simulink model "Slope_Road_SideSlipAngle_Vx_Estimation"  (R2024b)
settings: Solver=FixedStepAuto  StartTime=0.0  StopTime=7.5  FixedStep=0.001  RelTol=1e-4
values from neighbouring files (symbols this model uses):
  ax_long_1 = 1    [Init.m]
  ax_long_2 = 3    [Init.m]
  ax_long_3 = 6    [Init.m]
  ax_steer_1 = 0.5    [Init.m]
  ax_steer_2 = 1.5    [Init.m]
  ax_steer_3 = 3    [Init.m]
  ax_vx_thres1 = 0.5    [Init.m]
  ax_vx_thres2 = 3    [Init.m]
  Brush = [28.93,1.496,0.9486,0.06054]    [Init.m]
  delay_constant = 1/delay_length*ones(1,round(delay_length))    [Init.m]
  delta_thres = 3*3.14/180    (= 0.0523333333333)    [Init.m]
  deltarate_thres = 0.1    [Init.m]
  dg2rd = pi/180    (= 0.0174532925199)    [Init.m]
  excessive_wheel_intgr = 1000    [Init.m]
  filter_ratio_ax_ay = 0.2    [Init.m]
  g = 9.8    [Init.m]
  gao_ay = 1.5    [Init.m]
  gao_D_v = 0.2    [Init.m]
  gao_D_w = 0.03    [Init.m]
  gao_D_w1 = 0.25    [Init.m]
  gao_gz = 0.1    [Init.m]
  gao_Q = 1e-02    (= 0.01)    [Init.m]
  gao_R = 0.00077574*0.1    (= 7.7574e-05)    [Init.m]
  K_theta = 1    [Init.m]
  k_vx_vari_thres1 = 20    [Init.m]
  k_vx_vari_thres2 = 20    [Init.m]
  k_vx_vari_thres3 = 20    [Init.m]
  k_vy = 1/veh_m0    (= 0.000327653997379)    [Init.m]
  N_num = 6    [Init.m]
  para_long_1 = 1    [Init.m]
  para_long_2 = 100    [Init.m]
  para_long_3 = 100000000    [Init.m]
  para_long_4 = 100    [Init.m]
  para_steer_1 = 0.1    [Init.m]
  para_steer_2 = 10    [Init.m]
  para_steer_3 = 1000    [Init.m]
  para_steer_4 = 1000    [Init.m]
  rd2dg = 180/pi    (= 57.2957795131)    [Init.m]
  Steer_angle = 0    [Init.m]
  tao_1 = 6    [Init.m]
  time_interval = 1/Ts    (= 1000)    [Init.m]
  Ts = 0.001    [Init.m]
  u_init = 0.9    [Init.m]
  veh_bf = 1.600    (= 1.6)    [Init.m]
  veh_br = 1.740    (= 1.74)    [Init.m]
  veh_lf = 1.293    [Init.m]
  veh_lr = veh_l-veh_lf    (= 1.835)    [Init.m]
  veh_m0 = 3052    [Init.m]
  vx_cri = 1    [Init.m]
  vx_lowest = 0.01    [Init.m]
  vx_max_diff = 1    [Init.m]
  vy_new_ini = 0    [Init.m]
  wh_r = 0.346    [Init.m]
undefined symbols (not defined in the file or in its folder): DiscIntNeverNeededParam, front_gear_ratio, rear_gear_ratio, steer_ratio
libraries: simulink x7, Solver_SF x1
(part 1 of 2)
settings Model: Creator=Lenovo  LastModifiedBy=13785
settings SolverCC: AlgebraicLoopSolver=TrustRegion
settings OptimizationCC: LifeSpan=inf
settings DebuggingCC: UnconnectedInputMsg=warning  UnconnectedOutputMsg=warning  UnconnectedLineMsg=warning  SFExecutionAtInitializationDiag=none  ArithmeticOperatorsInVariantConditions=warning
settings ModelReferenceCC: EnableRefExpFcnMdlSchedulingChecks=on
settings SFSimCC: CustomCodeUndefinedFunction=UseInterfaceOnly
settings RTWCC: GPUComputeCapability=3.5
settings CodeAppCC: StateflowObjectComments=on

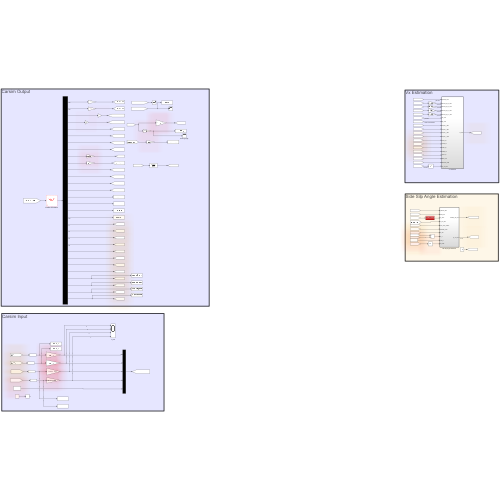
[thumbnail: Simulink's stored preview of the top-level diagram]
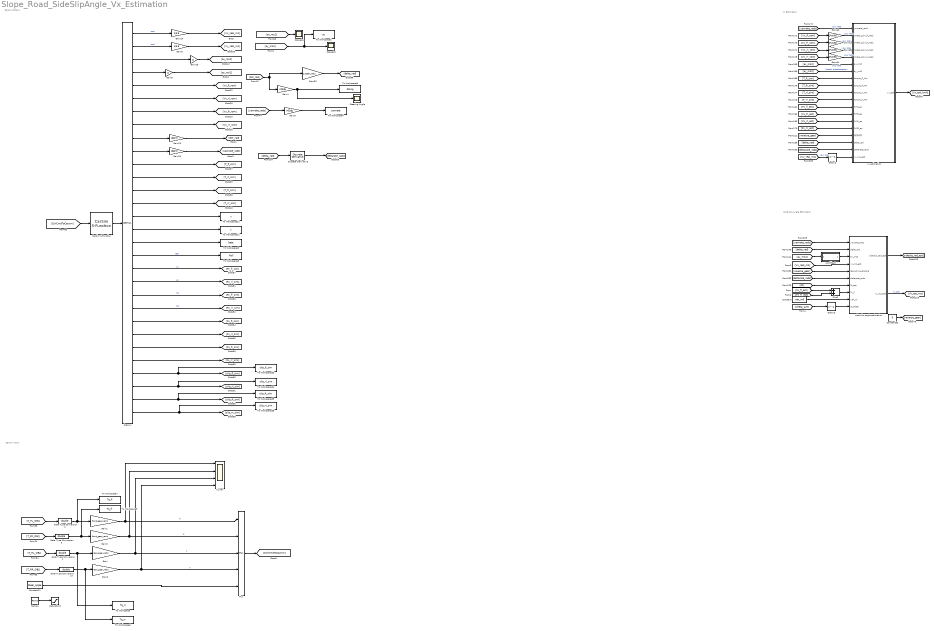
== system Slope_Road_SideSlipAngle_Vx_Estimation ==
  note: Vx Estimation
  note: Side Silp Angle Estimation
  note: Carsim Input
  note: Carsim Output
  CarSim S-Function : Solver_SF/CarSim S-Function  Priority=1  SIMFILE=simfile.sim  Run_RTs=off  vs_state_ind=Run  StopMode_ind=Vehicle Model
  Constant : Constant  Value=veh_m0
  Constant11 : Constant  Value=Steer_angle
  Constant32 : Constant  Value=0
  Data Type Conversion{1..3,27} (4 alike) : DataTypeConversion  OutDataTypeStr=double  SaturateOnIntegerOverflow=off  RndMeth=Floor
  Delay2 : Delay  DelayLength=1
  Delay3 : Delay  DelayLength=1  InitialCondition=u_init
  Demux : Demux  Outputs=30
  Discrete Derivative : simulink/Discrete/Discrete Derivative  gainval=1.0  ICPrevScaledInput=0.0  OutMin=[]  OutMax=[]  OutDataType=fixdt(1, 16)  OutScaling=2^-10  DoSatur=off
  Gain : Gain  Gain=rear_gear_ratio
  Gain1 : Gain  Gain=front_gear_ratio
  Gain2 : Gain  Gain=rear_gear_ratio
  Gain24 : Gain  Gain=1/3.6
  Gain25 : Gain  Gain=dg2rd
  Gain26 : Gain  Gain=dg2rd
  Gain29 : Gain  Gain=g
  Gain3 : Gain  Gain=front_gear_ratio
  Gain4 : Gain  Gain=rd2dg
  Gain5 : Gain  Gain=rd2dg
  Gain53 : Gain  Gain=1/steer_ratio
  Gain6 : Gain  Gain=1/3.6
  Gain{60..61,63..64} (4 alike) : Gain  Gain=2*pi/60
  Gain8 : Gain  Gain=g
  Mux : Mux  Inputs=5
  Plus2 : Sum
  Ramp1 : simulink/Sources/Ramp  slope=500  start=1  InitialOutput=0
  Saturation1 : Saturate  UpperLimit=300
  Scope10 : Scope
  Scope16 : Scope
  Steering Angle : Scope
  T_final : Scope  NumInputPorts=4
  To Workspace : ToWorkspace  VariableName=Tq_rl  SaveFormat=Timeseries  SampleTime=-1
  To Workspace11 : ToWorkspace  VariableName=x  SaveFormat=Timeseries  SampleTime=-1
  To Workspace12 : ToWorkspace  VariableName=y  SaveFormat=Timeseries  SampleTime=-1
  To Workspace2 : ToWorkspace  VariableName=ay  SaveFormat=Timeseries  SampleTime=-1
  To Workspace3 : ToWorkspace  VariableName=StAng  SaveFormat=Timeseries  SampleTime=-1
  To Workspace33 : ToWorkspace  VariableName=slip_fl_sim  SaveFormat=Timeseries  SampleTime=-1
  To Workspace34 : ToWorkspace  VariableName=slip_rl_sim  SaveFormat=Timeseries  SampleTime=-1
  To Workspace35 : ToWorkspace  VariableName=slip_fr_sim  SaveFormat=Timeseries  SampleTime=-1
  To Workspace36 : ToWorkspace  VariableName=slip_rr_sim  SaveFormat=Timeseries  SampleTime=-1
  To Workspace4 : ToWorkspace  VariableName=yawrate  SaveFormat=Timeseries  SampleTime=-1
  To Workspace5 : ToWorkspace  VariableName=beta  SaveFormat=Timeseries  SampleTime=-1
  To Workspace6 : ToWorkspace  VariableName=Tq_rr  SaveFormat=Timeseries  SampleTime=-1
  To Workspace7 : ToWorkspace  VariableName=Tq_fl  SaveFormat=Timeseries  SampleTime=-1
  To Workspace8 : ToWorkspace  VariableName=Roll  SaveFormat=Timeseries  SampleTime=-1
  To Workspace9 : ToWorkspace  VariableName=Tq_fr  SaveFormat=Timeseries  SampleTime=-1
  rpmfilter3 : Subsystem
  "side slip angle estimation " : Subsystem  TreatAsAtomicUnit=on
  vx estimation : Subsystem  TreatAsAtomicUnit=on
  wires:
  "side slip angle estimation "/2(vy_ms_esti) -> [Vy_est_ms]  "vy_est"
  [Fx_fl_est] -> Plus2/1
  [yawrate_rads] -> "side slip angle estimation "/1(yawrate_rads)
  Plus2/1 -> "side slip angle estimation "/8(Fx_f)
  [reverse_gear] -> "side slip angle estimation "/5(rear_drive_enable)
  [Fx_fr_est] -> Plus2/2
  "side slip angle estimation "/1(sideslip_rad_esti) -> [sideslip_rad_esti]
  [Fz] -> "side slip angle estimation "/7(Fz_est)
  [delta_rad] -> "side slip angle estimation "/2(delta_rad)
  rpmfilter3/1(fliter_out) -> "side slip angle estimation "/3(ay_ms2)
  [deltarate_rads] -> "side slip angle estimation "/6(deltarate_rads)
  [ay_ms2] -> rpmfilter3/1(fliter_in)
  Constant/1 -> "side slip angle estimation "/9(veh_m)
  Delay3/1 -> "side slip angle estimation "/10(rd_theta)
  Constant32/1 -> [reverse_gear]
  [deltarate_rads] -> vx estimation/18(deltarate_rads)
  [Vx_rl_rpm] -> Gain63/1
  Gain61/1 -> vx estimation/3(wheel_spin_fr_rads)  "yaw rate"
  Delay2/1 -> vx estimation/19(vy_ms_esti)
  [T_rl_sim] -> vx estimation/10(torque_rl_Nm)
  [Fx_fr_est] -> vx estimation/13(FxFR_es)
  [Vy_real_ms] -> Delay2/1  "yaw rate"
  [Vx_fr_rpm] -> Gain61/1
  [T_fl_sim] -> vx estimation/8(torque_fl_Nm)
  [Vx_fl_rpm] -> Gain60/1
  Gain63/1 -> vx estimation/4(wheel_spin_rl_rads)  "yaw rate"
  [reverse_gear] -> vx estimation/16(倒挡信息)
  [yawrate_rads] -> vx estimation/1(yawrate_rads)  "yaw rate"
  Gain64/1 -> vx estimation/5(wheel_spin_rr_rads)  "yaw rate"
  Gain60/1 -> vx estimation/2(wheel_spin_fl_rads)  "yaw rate"
  [ax_ms2] -> vx estimation/6(ax_ms2)  "yaw rate"
  [delta_rad] -> vx estimation/17(delta_rad)
  vx estimation/1(vx_esti) -> [Vx_est_kmh]
  [Fx_fl_est] -> vx estimation/12(FxFL_es)
  [ay_ms2] -> vx estimation/7(ay_ms2)  "lateral acceleratation"
  [Fx_rr_est] -> vx estimation/15(FxRR_es)
  [T_rr_sim] -> vx estimation/11(torque_rr_Nm)
  [Fx_rl_est] -> vx estimation/14(FxRL_es)
  [Vx_rr_rpm] -> Gain64/1
  [T_fr_sim] -> vx estimation/9(torque_fr_Nm)
  [Vx_real_ms] -> "side slip angle estimation "/4(vx_ms_esti)
  [theta_ave] -> Delay3/1
  Gain29/1 -> [ax_ms2]
  Gain1/1 -> T_final/1, Mux/1  "fl"
  Demux/2 -> Gain6/1  "real"
  Demux/26 -> [Fx_rr_sim]
  [CtrlCmdToCarsim] -> CarSim S-Function/1
  Demux/12 -> [T_rl_sim]
  Demux/5 -> [Vx_fl_rpm]
  [ax_ms2] -> Scope16/1
  [delta_rad] -> Discrete Derivative/1
  Gain5/1 -> To Workspace4/1
  CarSim S-Function/1 -> Demux/1
  Demux/7 -> [Vx_fr_rpm]
  [T_FR_OBJ] -> Data Type Conversion3/1
  Demux/30 -> [slip_rr_sim], To Workspace36/1
  Demux/11 -> [T_fl_sim]
  Mux/1 -> [CtrlCmdToCarsim]
  Demux/10 -> Gain26/1
  Gain26/1 -> [yawrate_rads]
  Data Type Conversion27/1 -> To Workspace6/1, Gain2/1
  Demux/29 -> [slip_fr_sim], To Workspace35/1
  Demux/4 -> Gain8/1
  [ay_ms2] -> Scope10/1, To Workspace2/1
  Gain8/1 -> [ay_ms2]
  Gain3/1 -> Mux/2, T_final/2  "fr"
  Demux/27 -> To Workspace33/1, [slip_fl_sim]
  Demux/1 -> Gain24/1  "real"
  Gain4/1 -> Steering Angle/1, To Workspace3/1
  Gain6/1 -> [Vy_real_ms]
  Data Type Conversion1/1 -> To Workspace/1, Gain/1
  Demux/28 -> [slip_rl_sim], To Workspace34/1
  Demux/9 -> Gain25/1
  Demux/8 -> [Vx_rr_rpm]
  Gain/1 -> Mux/3, T_final/3  "rl"
  Constant11/1 -> Mux/5
  Data Type Conversion2/1 -> To Workspace7/1, Gain1/1
  Demux/13 -> [T_fr_sim]
  [T_RL_OBJ] -> Data Type Conversion1/1
  [T_RR_OBJ] -> Data Type Conversion27/1
  Demux/3 -> Gain29/1
  Gain24/1 -> [Vx_real_ms]
  Demux/6 -> [Vx_rl_rpm]
  Gain2/1 -> Mux/4, T_final/4  "rr"
  Gain25/1 -> [SW_rad]
  Demux/14 -> [T_rr_sim]
  Gain53/1 -> [delta_rad]
  Discrete Derivative/1 -> [deltarate_rads]
  [SW_rad] -> Gain4/1, Gain53/1
  Data Type Conversion3/1 -> To Workspace9/1, Gain3/1
  Ramp1/1 -> Saturation1/1
  [yawrate_rads] -> Gain5/1
  [T_FL_OBJ] -> Data Type Conversion2/1
  Demux/19 -> [Fz_fl_sim]  "L1"
  Demux/20 -> [Fz_rl_sim]  "L2"
  Demux/21 -> [Fz_fr_sim]  "R1"
  Demux/22 -> [Fz_rr_sim]  "R2"
  Demux/25 -> [Fx_fr_sim]
  Demux/24 -> [Fx_rl_sim]
  Demux/23 -> [Fx_fl_sim]
  Demux/15 -> To Workspace11/1
  Demux/16 -> To Workspace12/1
  Demux/17 -> To Workspace5/1
  Demux/18 -> To Workspace8/1  "real"

== system Slope_Road_SideSlipAngle_Vx_Estimation/rpmfilter3 ==
  fliter_in : Inport
  Constant1 : Constant  OutDataTypeStr=single
  Divide : Product  Inputs=**
  Divide1 : Product  Inputs=**
  Sum : Sum  Inputs=|-+
  Sum1 : Sum  Inputs=|++
  Unit Delay : UnitDelay  SampleTime=-1  HasFrameUpgradeWarning=on
  afa : Constant  Value=filter_ratio_ax_ay  OutDataTypeStr=single
  fliter_out : Outport
  wires:
  Unit Delay/1 -> Divide1/2
  fliter_in/1 -> Divide/1
  Divide1/1 -> Sum1/2
  Divide/1 -> Sum1/1
  Sum/1 -> Divide1/1
  afa/1 -> Divide/2, Sum/1
  Constant1/1 -> Sum/2
  Sum1/1 -> Unit Delay/1, fliter_out/1

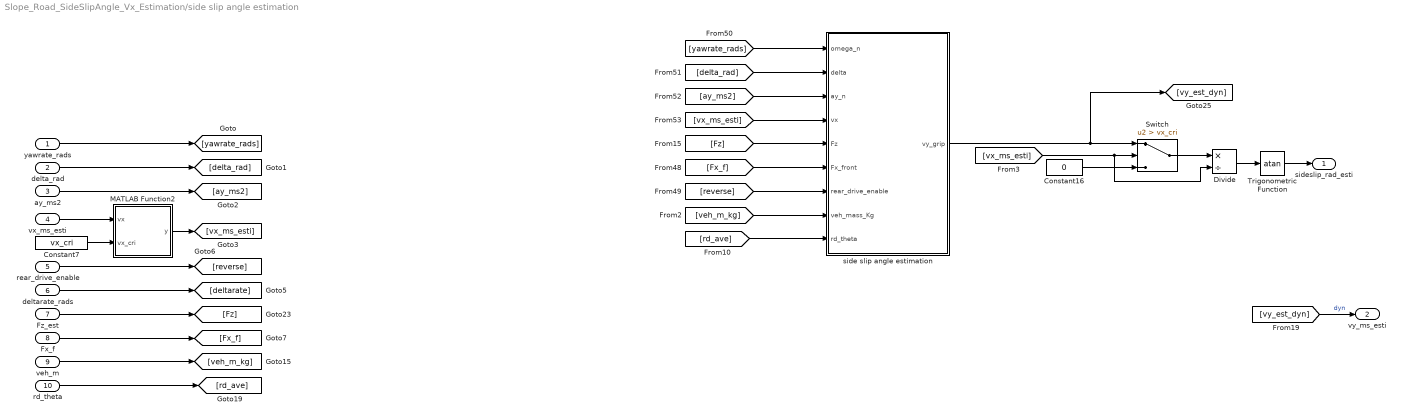
== system Slope_Road_SideSlipAngle_Vx_Estimation/side slip angle estimation  ==
  yawrate_rads : Inport
  delta_rad : Inport  Port=2
  ay_ms2 : Inport  Port=3
  vx_ms_esti : Inport  Port=4
  rear_drive_enable : Inport  Port=5
  deltarate_rads : Inport  Port=6
  Fz_est : Inport  Port=7
  Fx_f : Inport  Port=8
  veh_m : Inport  Port=9
  rd_theta : Inport  Port=10
  Constant16 : Constant  Value=0
  Constant7 : Constant  Value=vx_cri
  Divide : Product  Inputs=*/
  MATLAB Function2 : MATLAB Function  TreatAsAtomicUnit=on
  Switch : Switch  Criteria=u2 > Threshold  Threshold=vx_cri  SaturateOnIntegerOverflow=off  InputSameDT=off
  Trigonometric Function : Trigonometry  Operator=atan
  side slip angle estimation : Subsystem  TreatAsAtomicUnit=on
  sideslip_rad_esti : Outport
  vy_ms_esti : Outport  Port=2
  wires:
  vx_ms_esti/1 -> MATLAB Function2/1(vx)
  MATLAB Function2/1(y) -> [vx_ms_esti]
  Constant7/1 -> MATLAB Function2/2(vx_cri)
  ay_ms2/1 -> [ay_ms2]
  yawrate_rads/1 -> [yawrate_rads]
  delta_rad/1 -> [delta_rad]
  Fz_est/1 -> [Fz]
  deltarate_rads/1 -> [deltarate]
  Fx_f/1 -> [Fx_f]
  veh_m/1 -> [veh_m_kg]
  rear_drive_enable/1 -> [reverse]
  rd_theta/1 -> [rd_ave]
  [yawrate_rads] -> side slip angle estimation/1(omega_n)
  [Fx_f] -> side slip angle estimation/6(Fx_front)
  [delta_rad] -> side slip angle estimation/2(delta)
  [vx_ms_esti] -> side slip angle estimation/4(vx)
  [ay_ms2] -> side slip angle estimation/3(ay_n)
  [Fz] -> side slip angle estimation/5(Fz)
  Constant16/1 -> Switch/3
  side slip angle estimation/1(vy_grip) -> [vy_est_dyn], Switch/1
  [vx_ms_esti] -> Divide/2, Switch/2
  Switch/1 -> Divide/1
  [veh_m_kg] -> side slip angle estimation/8(veh_mass_Kg)
  Trigonometric Function/1 -> sideslip_rad_esti/1
  [rd_ave] -> side slip angle estimation/9(rd_theta)
  Divide/1 -> Trigonometric Function/1
  [vy_est_dyn] -> vy_ms_esti/1  "dyn"
  [reverse] -> side slip angle estimation/7(rear_drive_enable)

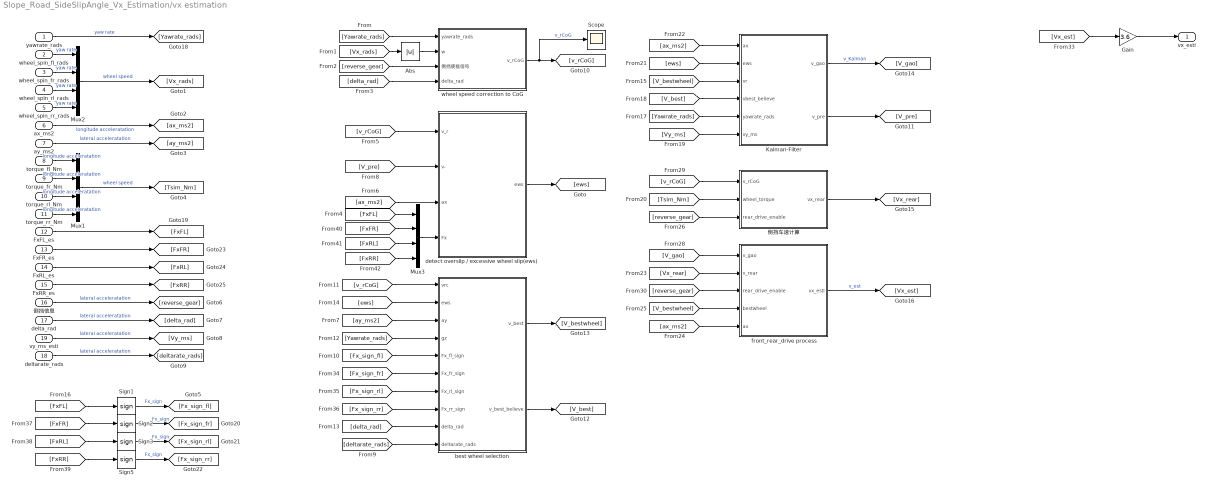
== system Slope_Road_SideSlipAngle_Vx_Estimation/vx estimation ==
  yawrate_rads : Inport
  wheel_spin_fl_rads : Inport  Port=2
  wheel_spin_fr_rads : Inport  Port=3
  wheel_spin_rl_rads : Inport  Port=4
  wheel_spin_rr_rads : Inport  Port=5
  ax_ms2 : Inport  Port=6
  ay_ms2 : Inport  Port=7
  torque_fl_Nm : Inport  Port=8
  torque_fr_Nm : Inport  Port=9
  torque_rl_Nm : Inport  Port=10
  torque_rr_Nm : Inport  Port=11
  FxFL_es : Inport  Port=12
  FxFR_es : Inport  Port=13
  FxRL_es : Inport  Port=14
  FxRR_es : Inport  Port=15
  倒挡信息 : Inport  Port=16
  delta_rad : Inport  Port=17
  deltarate_rads : Inport  Port=18
  vy_ms_esti : Inport  Port=19
  Abs : Abs  SaturateOnIntegerOverflow=off
  Gain : Gain  Gain=3.6
  Kalman-Filter : Subsystem
  Mux1 : Mux
  Mux2 : Mux
  Mux3 : Mux
  Scope : Scope
  Sign{1..3,5} (4 alike) : Signum
  "best wheel selection " : Subsystem
  detect overslip / excessive wheel slip(ews) : Subsystem
  front_rear_drive process : Subsystem  TreatAsAtomicUnit=on
  wheel speed correction to CoG : Subsystem
  倒挡车速计算 : Subsystem  TreatAsAtomicUnit=on
  vx_esti : Outport
  wires:
  vy_ms_esti/1 -> [Vy_ms]  "lateral acceleratation"
  torque_rr_Nm/1 -> Mux1/4  "longitude acceleratation"
  torque_rl_Nm/1 -> Mux1/3  "longitude acceleratation"
  torque_fr_Nm/1 -> Mux1/2  "longitude acceleratation"
  torque_fl_Nm/1 -> Mux1/1  "longitude acceleratation"
  wheel_spin_rr_rads/1 -> Mux2/4  "yaw rate"
  wheel_spin_rl_rads/1 -> Mux2/3  "yaw rate"
  wheel_spin_fr_rads/1 -> Mux2/2  "yaw rate"
  wheel_spin_fl_rads/1 -> Mux2/1  "yaw rate"
  yawrate_rads/1 -> [Yawrate_rads]  "yaw rate"
  Mux2/1 -> [Vx_rads]  "wheel speed"
  ax_ms2/1 -> [ax_ms2]  "longitude acceleratation"
  ay_ms2/1 -> [ay_ms2]  "lateral acceleratation"
  Mux1/1 -> [Tsim_Nm]  "wheel speed"
  FxFL_es/1 -> [FxFL]
  倒挡信息/1 -> [reverse_gear]  "lateral acceleratation"
  delta_rad/1 -> [delta_rad]  "lateral acceleratation"
  deltarate_rads/1 -> [deltarate_rads]  "lateral acceleratation"
  [Vx_rads] -> Abs/1
  [Yawrate_rads] -> wheel speed correction to CoG/1(yawrate_rads)
  wheel speed correction to CoG/1(v_rCoG) -> Scope/1, [v_rCoG]  "v_rCoG"
  [delta_rad] -> wheel speed correction to CoG/4(delta_rad)
  [reverse_gear] -> wheel speed correction to CoG/3(倒挡使能信号)
  Abs/1 -> wheel speed correction to CoG/2(w)
  [v_rCoG] -> detect overslip / excessive wheel slip(ews)/1(v_r)
  [ax_ms2] -> detect overslip / excessive wheel slip(ews)/3(ax)
  [V_pre] -> detect overslip / excessive wheel slip(ews)/2(v-)
  detect overslip / excessive wheel slip(ews)/1(ews) -> [ews]
  "best wheel selection "/2(v_best_believe) -> [V_best]
  [v_rCoG] -> "best wheel selection "/1(vrc)
  "best wheel selection "/1(v_best) -> [V_bestwheel]
  [Yawrate_rads] -> "best wheel selection "/4(gz)
  [delta_rad] -> "best wheel selection "/9(delta_rad)
  [deltarate_rads] -> "best wheel selection "/10(deltarate_rads)
  [ay_ms2] -> "best wheel selection "/3(ay)
  [ews] -> "best wheel selection "/2(ews)
  [Yawrate_rads] -> Kalman-Filter/5(yawrate_rads)
  [Vy_ms] -> Kalman-Filter/6(vy_ms)
  [V_bestwheel] -> Kalman-Filter/3(vr)
  [ax_ms2] -> Kalman-Filter/1(ax)
  [V_best] -> Kalman-Filter/4(vbest_believe)
  [ews] -> Kalman-Filter/2(ews)
  Kalman-Filter/2(v_pre) -> [V_pre]
  Kalman-Filter/1(v_gao) -> [V_gao]  "v_Kalman"
  [reverse_gear] -> 倒挡车速计算/3(rear_drive_enable)
  [v_rCoG] -> 倒挡车速计算/1(v_rCoG)
  [ax_ms2] -> front_rear_drive process/5(ax)
  [reverse_gear] -> front_rear_drive process/3(rear_drive_enable)
  [Tsim_Nm] -> 倒挡车速计算/2(wheel_torque)
  [V_bestwheel] -> front_rear_drive process/4(bestwheel)
  [V_gao] -> front_rear_drive process/1(v_gao)
  倒挡车速计算/1(vx_rear) -> [Vx_rear]
  [Vx_rear] -> front_rear_drive process/2(v_rear)
  front_rear_drive process/1(vx_esti) -> [Vx_est]  "v_est"
  [Vx_est] -> Gain/1
  Gain/1 -> vx_esti/1
  Mux3/1 -> detect overslip / excessive wheel slip(ews)/4(Fx)
  Sign1/1 -> [Fx_sign_fl]  "Fx_sign"
  Sign2/1 -> [Fx_sign_fr]  "Fx_sign"
  Sign3/1 -> [Fx_sign_rl]  "Fx_sign"
  Sign5/1 -> [Fx_sign_rr]  "Fx_sign"
  [Fx_sign_fl] -> "best wheel selection "/5(Fx_fl_sign)
  [Fx_sign_fr] -> "best wheel selection "/6(Fx_fr_sign)
  [Fx_sign_rl] -> "best wheel selection "/7(Fx_rl_sign)
  [Fx_sign_rr] -> "best wheel selection "/8(Fx_rr_sign)
  FxFR_es/1 -> [FxFR]
  FxRL_es/1 -> [FxRL]
  FxRR_es/1 -> [FxRR]
  [FxFL] -> Sign1/1
  [FxFR] -> Sign2/1
  [FxRL] -> Sign3/1
  [FxRR] -> Sign5/1
  [FxFR] -> Mux3/2
  [FxFL] -> Mux3/1
  [FxRL] -> Mux3/3
  [FxRR] -> Mux3/4

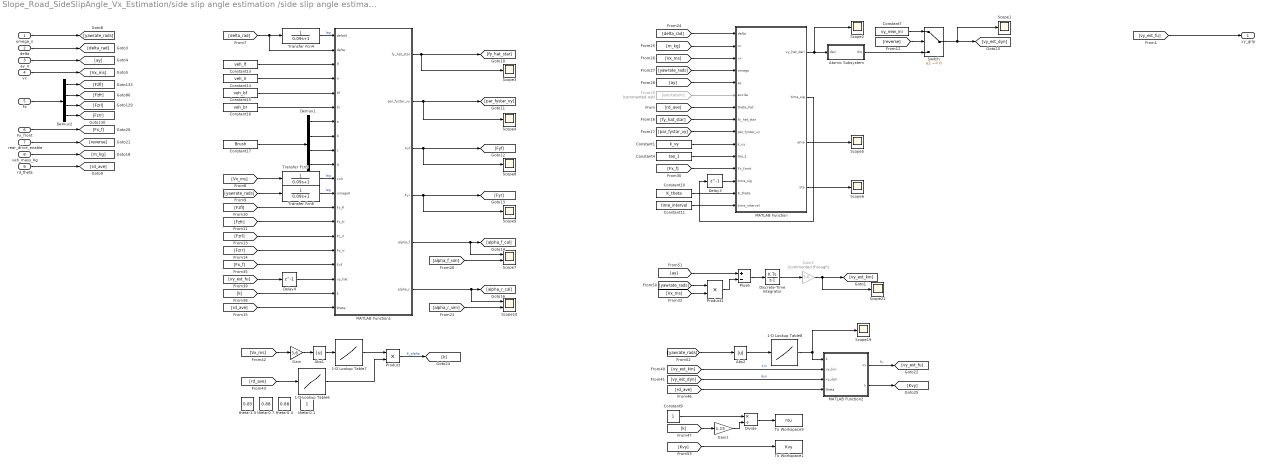
== system Slope_Road_SideSlipAngle_Vx_Estimation/side slip angle estimation /side slip angle estimation ==
  omega_n : Inport
  delta : Inport  Port=2
  ay_n : Inport  Port=3
  vx : Inport  Port=4
  Fz : Inport  Port=5
  Fx_front : Inport  Port=6
  rear_drive_enable : Inport  Port=7
  veh_mass_Kg : Inport  Port=8
  rd_theta : Inport  Port=9
  1-D Lookup Table6 : Lookup_n-D  NumberOfTableDimensions=1  BreakpointsForDimension1=[0 0.4 0.7 1.0 1.1]  Table=[0.93 0.92 0.92 0.91 0.91]  InternalRulePriority=Speed  RndMeth=Simplest
  1-D Lookup Table7 : Lookup_n-D  NumberOfTableDimensions=1  BreakpointsForDimension1=[0 50 60 70 80]  Table=[1.08 1.08 1.08 1.09 1.13]*1.15  InternalRulePriority=Speed  RndMeth=Simplest
  1-D Lookup Table8 : Lookup_n-D  NumberOfTableDimensions=1  BreakpointsForDimension1=[0 0.4 0.5 0.6 0.8]  Table=[0.9 0.9 0.4 0.1 0.1]  InternalRulePriority=Speed  RndMeth=Simplest
  Abs1 : Abs  SaturateOnIntegerOverflow=off
  Abs2 : Abs  SaturateOnIntegerOverflow=off
  Atomic Subsystem : Subsystem  TreatAsAtomicUnit=on
  Constant1 : Constant  Value=k_vy
  Constant10 : Constant  Value=K_theta
  Constant11 : Constant  Value=time_interval
  Constant13 : Constant  Value=veh_lf
  Constant14 : Constant  Value=veh_lr
  Constant15 : Constant  Value=veh_bf
  Constant16 : Constant  Value=veh_br
  Constant17 : Constant  Value=Brush
  Constant4 : Constant  Value=tao_1
  Constant7 : Constant  Value=vy_new_ini
  Constant9 : Constant
  Delay3 : Delay  DelayLength=1
  Delay4 : Delay  DelayLength=1
  Demux1 : Demux
  Demux2 : Demux
  Discrete-Time Integrator : DiscreteIntegrator  SampleTime=-1  ICPrevOutput=DiscIntNeverNeededParam  ICPrevScaledInput=DiscIntNeverNeededParam
  Divide : Product  Inputs=*/
  From29 : From  Commented=on  GotoTag=excitation
  Gain : Gain  Gain=3.6
  Gain1 : Gain  Gain=1.15
  Gain3 : Gain  Commented=through  Gain=3.6
  MATLAB Function : MATLAB Function  TreatAsAtomicUnit=on
  MATLAB Function1 : MATLAB Function  TreatAsAtomicUnit=on
  MATLAB Function2 : MATLAB Function  TreatAsAtomicUnit=on
  Plus6 : Sum  Inputs=+-
  Product : Product
  Product1 : Product
  Scope{1..6,8..9,19,22} (10 alike) : Scope
  Scope10 : Scope  NumInputPorts=2
  Scope7 : Scope  NumInputPorts=2
  Switch : Switch  Criteria=u2 ~= 0  SaturateOnIntegerOverflow=off  InputSameDT=off
  To Workspace1 : ToWorkspace  VariableName=Kvy  SampleTime=-1
  To Workspace9 : ToWorkspace  VariableName=rou  SampleTime=-1
  Transfer Fcn4 : TransferFcn  Denominator=[0.09 1]
  Transfer Fcn5 : TransferFcn  Denominator=[0.09 1]
  Transfer Fcn6 : TransferFcn  Denominator=[0.09 1]
  theta-0.1 : Constant
  theta-0.4 : Constant  Value=0.88
  theta-0.7 : Constant  Value=0.88
  theta-1.0 : Constant  Value=0.85
  vy_grip : Outport
  wires:
  [delta_rad] -> MATLAB Function/1(delta)
  [Vx_ms] -> MATLAB Function/3(vx)
  [m_kg] -> MATLAB Function/2(m)
  [ay] -> MATLAB Function/5(ay)
  [yawrate_rads] -> MATLAB Function/4(omega)
  MATLAB Function/1(vy_hat_deri) -> Scope2/1, Atomic Subsystem/1(deri)
  Constant1/1 -> MATLAB Function/10(k_vy)
  Constant4/1 -> MATLAB Function/11(tao_1)
  [Fx_f] -> MATLAB Function/12(Fx_front)
  Constant10/1 -> MATLAB Function/14(K_theta)
  MATLAB Function/2(time_sig) -> Delay3/1
  Constant11/1 -> MATLAB Function/15(time_interval)
  Constant7/1 -> Switch/1
  Atomic Subsystem/1(rho) -> Switch/3
  Switch/1 -> Scope1/1, [vy_est_dyn]
  [delta_rad] -> Transfer Fcn4/1, MATLAB Function1/2(delta)
  Transfer Fcn4/1 -> MATLAB Function1/1(delta0)  "lag"
  Constant13/1 -> MATLAB Function1/3(lf)
  Constant14/1 -> MATLAB Function1/4(lr)
  Constant15/1 -> MATLAB Function1/5(bf)
  Constant16/1 -> MATLAB Function1/6(br)
  Constant17/1 -> Demux1/1
  Demux1/1 -> MATLAB Function1/7(a)
  Demux1/2 -> MATLAB Function1/8(b)
  Demux1/3 -> MATLAB Function1/9(c)
  Demux1/4 -> MATLAB Function1/10(d)
  vx/1 -> [Vx_ms]
  Transfer Fcn5/1 -> MATLAB Function1/11(vx0)  "lag"
  Transfer Fcn6/1 -> MATLAB Function1/12(omega0)  "lag"
  [Fzfl] -> MATLAB Function1/13(Fz_fl)
  MATLAB Function1/2(par_fystar_vy) -> Scope4/1, [par_fystar_vy]
  MATLAB Function1/3(Fyf) -> Scope8/1, [Fyf]
  MATLAB Function1/4(Fyr) -> Scope9/1, [Fyr]
  MATLAB Function1/1(fy_hat_star) -> Scope3/1, [fy_hat_star]
  MATLAB Function/3(ema) -> Scope5/1
  MATLAB Function/4(ota) -> Scope6/1
  [vy_est_fu] -> Delay4/1
  MATLAB Function1/5(alpha_f) -> Scope7/1, [alpha_f_cal]
  delta/1 -> [delta_rad]
  [Vx_ms] -> Transfer Fcn5/1
  omega_n/1 -> [yawrate_rads]
  [yawrate_rads] -> Transfer Fcn6/1
  Demux2/2 -> [Fzfr]
  Demux2/3 -> [Fzrl]
  Demux2/1 -> [Fzfl]
  Fz/1 -> Demux2/1
  Demux2/4 -> [Fzrr]
  [Fzfr] -> MATLAB Function1/14(Fz_fr)
  [Fzrl] -> MATLAB Function1/15(Fz_rl)
  [Fzrr] -> MATLAB Function1/16(Fz_rr)
  rd_theta/1 -> [rd_ave]
  [fy_hat_star] -> MATLAB Function/8(fy_hat_star)
  [par_fystar_vy] -> MATLAB Function/9(par_fystar_vy)
  MATLAB Function1/6(alpha_r) -> Scope10/1, [alpha_r_cal]
  [alpha_f_sim] -> Scope7/2
  [alpha_r_sim] -> Scope10/2
  veh_mass_Kg/1 -> [m_kg]
  ay_n/1 -> [ay]
  From29/1 -> MATLAB Function/6(excita)
  Fx_front/1 -> [Fx_f]
  Delay3/1 -> MATLAB Function/13("time_sig ")
  rear_drive_enable/1 -> [reverse]
  [reverse] -> Switch/2
  Delay4/1 -> MATLAB Function1/18(vy_hat)
  [rd_ave] -> MATLAB Function/7(theta_hat)
  [vy_est_fu] -> vy_grip/1
  [k] -> MATLAB Function1/19(k)
  [rd_ave] -> MATLAB Function1/20(theta)
  [Fx_f] -> MATLAB Function1/17(Fxf)
  1-D Lookup Table7/1 -> Product/1
  Abs1/1 -> 1-D Lookup Table7/1
  Gain/1 -> Abs1/1
  Product/1 -> [k]  "K_alpha"
  1-D Lookup Table6/1 -> Product/2
  [Vx_ms] -> Gain/1
  [rd_ave] -> 1-D Lookup Table6/1
  [vy_est_kin] -> MATLAB Function2/2(vy_kin)  "kin"
  MATLAB Function2/2(k) -> [Kvy]
  [vy_est_dyn] -> MATLAB Function2/3(vy_dyn)  "dyn"
  [rd_ave] -> MATLAB Function2/4(theta)
  MATLAB Function2/1(vy) -> [vy_est_fu]  "fu"
  [yawrate_rads] -> Product1/1
  Plus6/1 -> Discrete-Time Integrator/1
  Discrete-Time Integrator/1 -> Gain3/1
  Product1/1 -> Plus6/2
  [ay] -> Plus6/1
  Gain3/1 -> Scope22/1, [vy_est_kin]
  [Vx_ms] -> Product1/2
  [yawrate_rads] -> Abs2/1
  Abs2/1 -> 1-D Lookup Table8/1
  1-D Lookup Table8/1 -> MATLAB Function2/1("k "), Scope19/1
  [k] -> Gain1/1
  [Kvy] -> To Workspace1/1
  Constant9/1 -> Divide/1
  Divide/1 -> To Workspace9/1
  Gain1/1 -> Divide/2

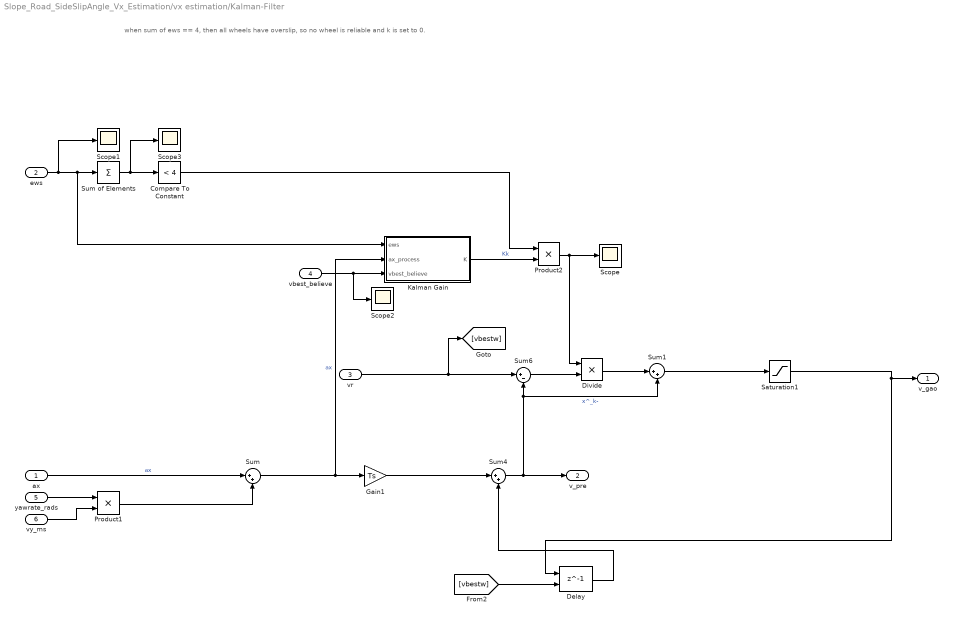
== system Slope_Road_SideSlipAngle_Vx_Estimation/vx estimation/Kalman-Filter ==
  note: when sum of ews == 4, then all wheels have overslip, so no wheel is reliable and k is set to 0.
  ax : Inport
  ews : Inport  Port=2
  vr : Inport  Port=3
  vbest_believe : Inport  Port=4
  yawrate_rads : Inport  Port=5
  vy_ms : Inport  Port=6
  Compare To Constant : simulink/Logic and Bit Operations/Compare To Constant  relop=<  const=4  OutDataTypeStr=uint8
  Delay : Delay  DelayLength=1  InitialConditionSource=Input port
      settings: InputPortMap=u0,p4
  Divide : Product  Inputs=**
  Gain1 : Gain  Gain=Ts
  Kalman Gain : Subsystem
  Product1 : Product
  Product2 : Product
  Saturation1 : Saturate  UpperLimit=1000  LowerLimit=0
  Scope{,1..3} (4 alike) : Scope
  Sum : Sum  Inputs=|++
  Sum of Elements : Sum  Inputs=+
  Sum1 : Sum  Inputs=|++
  Sum4 : Sum  Inputs=|++
  Sum6 : Sum  Inputs=|+-
  v_gao : Outport
  v_pre : Outport  Port=2
  wires:
  Saturation1/1 -> v_gao/1, Delay/1
  Product2/1 -> Scope/1, Divide/1
  Kalman Gain/1(K) -> Product2/2  "Kk"
  Product1/1 -> Sum/2
  vy_ms/1 -> Product1/2
  yawrate_rads/1 -> Product1/1
  vbest_believe/1 -> Kalman Gain/3(vbest_believe), Scope2/1
  Sum1/1 -> Saturation1/1
  [vbestw] -> Delay/2
  ax/1 -> Sum/1  "ax"
  vr/1 -> [vbestw], Sum6/1
  Sum of Elements/1 -> Compare To Constant/1, Scope3/1
  Sum4/1 -> Sum1/2, Sum6/2, v_pre/1  "x^_k-"
  Compare To Constant/1 -> Product2/1
  Gain1/1 -> Sum4/1
  Divide/1 -> Sum1/1
  Sum6/1 -> Divide/2
  Delay/1 -> Sum4/2
  ews/1 -> Scope1/1, Sum of Elements/1, Kalman Gain/1(ews)
  Sum/1 -> Kalman Gain/2(ax_process), Gain1/1  "ax"

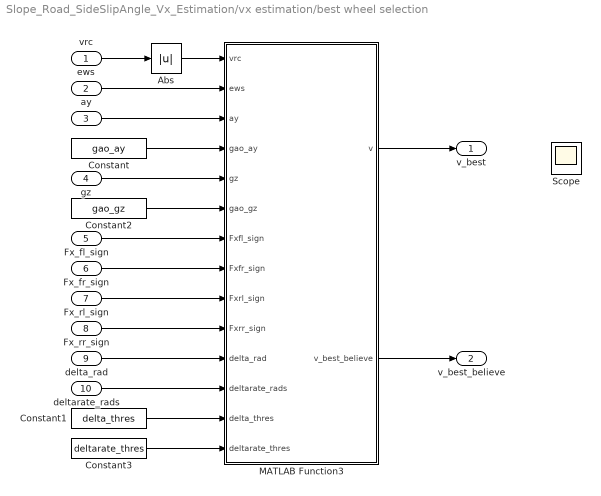
== system Slope_Road_SideSlipAngle_Vx_Estimation/vx estimation/best wheel selection  ==
  vrc : Inport
  ews : Inport  Port=2
  ay : Inport  Port=3
  gz : Inport  Port=4
  Fx_fl_sign : Inport  Port=5
  Fx_fr_sign : Inport  Port=6
  Fx_rl_sign : Inport  Port=7
  Fx_rr_sign : Inport  Port=8
  delta_rad : Inport  Port=9
  deltarate_rads : Inport  Port=10
  Abs : Abs  SaturateOnIntegerOverflow=off
  Constant : Constant  Value=gao_ay
  Constant1 : Constant  Value=delta_thres
  Constant2 : Constant  Value=gao_gz
  Constant3 : Constant  Value=deltarate_thres
  MATLAB Function3 : MATLAB Function  TreatAsAtomicUnit=on
  Scope : Scope
  v_best : Outport
  v_best_believe : Outport  Port=2
  wires:
  MATLAB Function3/2(v_best_believe) -> v_best_believe/1
  MATLAB Function3/1(v) -> v_best/1
  Constant2/1 -> MATLAB Function3/6(gao_gz)
  vrc/1 -> Abs/1
  ews/1 -> MATLAB Function3/2(ews)
  Abs/1 -> MATLAB Function3/1(vrc)
  Constant/1 -> MATLAB Function3/4(gao_ay)
  gz/1 -> MATLAB Function3/5(gz)
  delta_rad/1 -> MATLAB Function3/11(delta_rad)
  deltarate_rads/1 -> MATLAB Function3/12(deltarate_rads)
  Constant1/1 -> MATLAB Function3/13(delta_thres)
  Constant3/1 -> MATLAB Function3/14(deltarate_thres)
  Fx_fl_sign/1 -> MATLAB Function3/7(Fxfl_sign)
  Fx_fr_sign/1 -> MATLAB Function3/8(Fxfr_sign)
  Fx_rl_sign/1 -> MATLAB Function3/9(Fxrl_sign)
  Fx_rr_sign/1 -> MATLAB Function3/10(Fxrr_sign)
  ay/1 -> MATLAB Function3/3(ay)

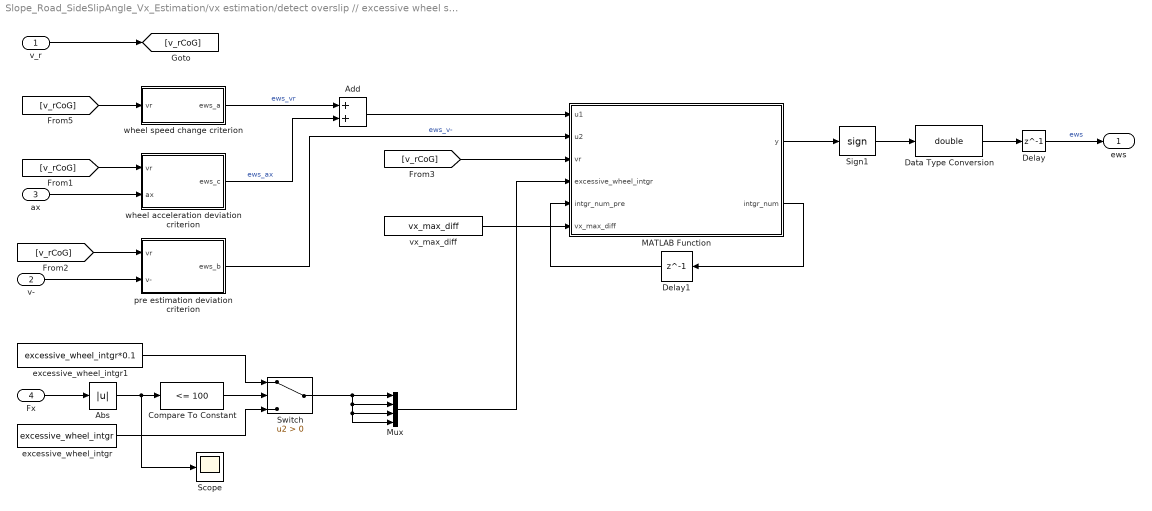
== system Slope_Road_SideSlipAngle_Vx_Estimation/vx estimation/detect overslip // excessive wheel slip(ews) ==
  v_r : Inport
  v- : Inport  Port=2
  ax : Inport  Port=3
  Fx : Inport  Port=4
  Abs : Abs  SaturateOnIntegerOverflow=off
  Add : Sum
  Compare To Constant : simulink/Logic and Bit Operations/Compare To Constant  relop=<=  const=100  OutDataTypeStr=boolean
  Data Type Conversion : DataTypeConversion  OutDataTypeStr=double  SaturateOnIntegerOverflow=off  RndMeth=Floor
  Delay : Delay  DelayLength=1
  Delay1 : Delay  DelayLength=1  InitialCondition=[0;0;0;0]
  MATLAB Function : MATLAB Function  TreatAsAtomicUnit=on
  Mux : Mux
  Scope : Scope
  Sign1 : Signum
  Switch : Switch  Criteria=u2 > Threshold  SaturateOnIntegerOverflow=off  InputSameDT=off
  excessive_wheel_intgr : Constant  Value=excessive_wheel_intgr
  excessive_wheel_intgr1 : Constant  Value=excessive_wheel_intgr*0.1
  pre estimation deviation criterion : Subsystem
  vx_max_diff : Constant  Value=vx_max_diff
  wheel acceleration deviation criterion : Subsystem
  wheel speed change criterion : Subsystem
  ews : Outport
  wires:
  pre estimation deviation criterion/1(ews_b) -> MATLAB Function/2(u2)  "ews_v-"
  Add/1 -> MATLAB Function/1(u1)
  MATLAB Function/2(intgr_num) -> Delay1/1
  vx_max_diff/1 -> MATLAB Function/6(vx_max_diff)
  Delay1/1 -> MATLAB Function/5(intgr_num_pre)
  MATLAB Function/1(y) -> Sign1/1
  ax/1 -> wheel acceleration deviation criterion/2(ax)
  wheel speed change criterion/1(ews_a) -> Add/1  "ews_vr"
  Delay/1 -> ews/1  "ews"
  wheel acceleration deviation criterion/1(ews_c) -> Add/2  "ews_ax"
  Data Type Conversion/1 -> Delay/1
  v-/1 -> pre estimation deviation criterion/2(v-)
  Sign1/1 -> Data Type Conversion/1
  [v_rCoG] -> wheel speed change criterion/1(vr)
  v_r/1 -> [v_rCoG]
  [v_rCoG] -> wheel acceleration deviation criterion/1(vr)
  [v_rCoG] -> pre estimation deviation criterion/1(vr)
  [v_rCoG] -> MATLAB Function/3(vr)
  Fx/1 -> Abs/1
  Compare To Constant/1 -> Switch/2
  excessive_wheel_intgr1/1 -> Switch/1
  excessive_wheel_intgr/1 -> Switch/3
  Abs/1 -> Scope/1, Compare To Constant/1
  Mux/1 -> MATLAB Function/4(excessive_wheel_intgr)
  Switch/1 -> Mux/2, Mux/3, Mux/4, Mux/1

== system Slope_Road_SideSlipAngle_Vx_Estimation/vx estimation/front_rear_drive process ==
  v_gao : Inport
  v_rear : Inport  Port=2
  rear_drive_enable : Inport  Port=3
  bestwheel : Inport  Port=4
  ax : Inport  Port=5
  Atomic Subsystem : Subsystem  TreatAsAtomicUnit=on
  Switch : Switch  Criteria=u2 ~= 0  SaturateOnIntegerOverflow=off  InputSameDT=off
  vx_esti : Outport
  wires:
  rear_drive_enable/1 -> Switch/2
  v_gao/1 -> Switch/3
  v_rear/1 -> Switch/1
  Atomic Subsystem/1(vx_esti) -> vx_esti/1
  Switch/1 -> Atomic Subsystem/1(vx)
  bestwheel/1 -> Atomic Subsystem/2(bestwheel)
  ax/1 -> Atomic Subsystem/3(ax)

== system Slope_Road_SideSlipAngle_Vx_Estimation/vx estimation/wheel speed correction to CoG ==
  yawrate_rads : Inport
  w : Inport  Port=2
  倒挡使能信号 : Inport  Port=3
  delta_rad : Inport  Port=4
  Constant1 : Constant  Value=-1
  Constant2 : Constant  Value=veh_lf
  Constant3 : Constant
  Gain1 : Gain  Gain=-veh_bf/2
  Gain2 : Gain  Gain=wh_r
  Gain3 : Gain  Gain=veh_bf/2
  Gain4 : Gain  Gain=veh_br/2
  Gain5 : Gain  Gain=-veh_br/2
  Mux : Mux
  Product : Product
  Switch : Switch  Criteria=u2 ~= 0  SaturateOnIntegerOverflow=off  InputSameDT=off
  yawrate_rads1 : InportShadow
  轮速到质心处车速 : MATLAB Function  TreatAsAtomicUnit=on
  v_rCoG : Outport
  wires:
  Constant2/1 -> 轮速到质心处车速/4(lf)
  delta_rad/1 -> 轮速到质心处车速/3(delta_rad)
  倒挡使能信号/1 -> Switch/2
  Product/1 -> Gain3/1, Gain1/1, Gain4/1, Gain5/1
  yawrate_rads/1 -> Product/1
  Switch/1 -> Product/2
  Constant3/1 -> Switch/3
  Constant1/1 -> Switch/1
  轮速到质心处车速/1(v_rCoG) -> v_rCoG/1
  w/1 -> Gain2/1
  Gain2/1 -> 轮速到质心处车速/1(u)
  yawrate_rads1/1 -> 轮速到质心处车速/5(yawrate_rads)
  Gain3/1 -> Mux/1
  Gain1/1 -> Mux/2
  Gain4/1 -> Mux/3
  Gain5/1 -> Mux/4
  Mux/1 -> 轮速到质心处车速/2(v)

== system Slope_Road_SideSlipAngle_Vx_Estimation/vx estimation/倒挡车速计算 ==
  v_rCoG : Inport
  wheel_torque : Inport  Port=2
  rear_drive_enable : Inport  Port=3
  MATLAB Function : MATLAB Function  TreatAsAtomicUnit=on
  vx_rear : Outport
  wires:
  v_rCoG/1 -> MATLAB Function/1(v_rCoG)
  MATLAB Function/1(vx_rear) -> vx_rear/1
  wheel_torque/1 -> MATLAB Function/2(wheel_torque)
  rear_drive_enable/1 -> MATLAB Function/3(rear_drive_enable)

== system Slope_Road_SideSlipAngle_Vx_Estimation/side slip angle estimation /side slip angle estimation/Atomic Subsystem ==
  deri : Inport
  Add : Sum
  Constant : Constant  Value=Ts
  Delay : Delay  DelayLength=1  InitialCondition=vy_new_ini
  Delay1 : Delay  DelayLength=1  InitialCondition=0
  Product1 : Product
  rho : Outport
  wires:
  Constant/1 -> Product1/2
  Add/1 -> Delay/1
  Product1/1 -> Add/2
  Delay/1 -> Add/1, rho/1
  deri/1 -> Delay1/1
  Delay1/1 -> Product1/1

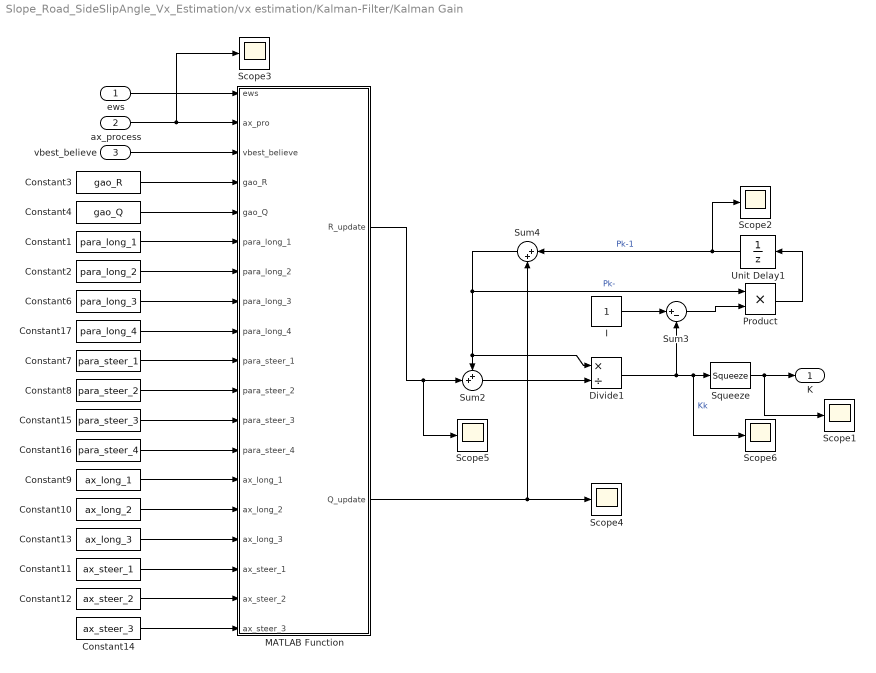
== system Slope_Road_SideSlipAngle_Vx_Estimation/vx estimation/Kalman-Filter/Kalman Gain ==
  ews : Inport
  ax_process : Inport  Port=2
  vbest_believe : Inport  Port=3
  Constant1 : Constant  Value=para_long_1
  Constant10 : Constant  Value=ax_long_2
  Constant11 : Constant  Value=ax_steer_1
  Constant12 : Constant  Value=ax_steer_2
  Constant13 : Constant  Value=ax_long_3
  Constant14 : Constant  Value=ax_steer_3
  Constant15 : Constant  Value=para_steer_3
  Constant16 : Constant  Value=para_steer_4
  Constant17 : Constant  Value=para_long_4
  Constant2 : Constant  Value=para_long_2
  Constant3 : Constant  Value=gao_R
  Constant4 : Constant  Value=gao_Q
  Constant6 : Constant  Value=para_long_3
  Constant7 : Constant  Value=para_steer_1
  Constant8 : Constant  Value=para_steer_2
  Constant9 : Constant  Value=ax_long_1
  Divide1 : Product  Inputs=*/
  I : Constant
  MATLAB Function : MATLAB Function  TreatAsAtomicUnit=on
  Product : Product
  Scope{1..6} (6 alike) : Scope
  Squeeze : Squeeze
  Sum2 : Sum  Inputs=++|
  Sum3 : Sum  Inputs=|+-
  Sum4 : Sum  Inputs=|++
  Unit Delay1 : UnitDelay  InitialCondition=1  SampleTime=-1  HasFrameUpgradeWarning=on
  K : Outport
  wires:
  Constant17/1 -> MATLAB Function/9(para_long_4)
  Constant16/1 -> MATLAB Function/13(para_steer_4)
  Constant15/1 -> MATLAB Function/12(para_steer_3)
  Constant14/1 -> MATLAB Function/19(ax_steer_3)
  Constant13/1 -> MATLAB Function/16(ax_long_3)
  Constant12/1 -> MATLAB Function/18(ax_steer_2)
  Constant11/1 -> MATLAB Function/17(ax_steer_1)
  Constant10/1 -> MATLAB Function/15(ax_long_2)
  Constant9/1 -> MATLAB Function/14(ax_long_1)
  Constant8/1 -> MATLAB Function/11(para_steer_2)
  Constant7/1 -> MATLAB Function/10(para_steer_1)
  Constant6/1 -> MATLAB Function/8(para_long_3)
  Constant2/1 -> MATLAB Function/7(para_long_2)
  Constant1/1 -> MATLAB Function/6(para_long_1)
  vbest_believe/1 -> MATLAB Function/3(vbest_believe)
  MATLAB Function/2(Q_update) -> Sum4/2, Scope4/1
  Constant4/1 -> MATLAB Function/5(gao_Q)
  Constant3/1 -> MATLAB Function/4(gao_R)
  ax_process/1 -> MATLAB Function/2(ax_pro), Scope3/1
  ews/1 -> MATLAB Function/1(ews)
  Divide1/1 -> Sum3/2, Scope6/1, Squeeze/1  "Kk"
  Sum2/1 -> Divide1/2
  I/1 -> Sum3/1
  Product/1 -> Unit Delay1/1
  Unit Delay1/1 -> Sum4/1, Scope2/1  "Pk-1"
  Sum4/1 -> Product/1, Divide1/1, Sum2/1  "Pk-"
  Squeeze/1 -> K/1, Scope1/1
  Sum3/1 -> Product/2
  MATLAB Function/1(R_update) -> Sum2/2, Scope5/1

== system Slope_Road_SideSlipAngle_Vx_Estimation/vx estimation/detect overslip // excessive wheel slip(ews)/pre estimation deviation criterion ==
  vr : Inport
  v- : Inport  Port=2
  Abs : Abs  SaturateOnIntegerOverflow=off
  Compare To Constant : simulink/Logic and Bit Operations/Compare To Constant  relop=>  const=gao_D_v  OutDataTypeStr=uint8
  Embedded MATLAB Function : MATLAB Function  TreatAsAtomicUnit=on
  Scope : Scope
  Scope1 : Scope
  Sum : Sum  Inputs=|+-
  Unit Delay : UnitDelay  SampleTime=-1  HasFrameUpgradeWarning=on
  gao_D_w : Constant  Value=gao_D_v
  ews_b : Outport
  wires:
  gao_D_w/1 -> Embedded MATLAB Function/2(gao_D_v)
  Abs/1 -> Scope/1, Embedded MATLAB Function/1(u)
  Embedded MATLAB Function/1(y) -> Unit Delay/1
  Unit Delay/1 -> Compare To Constant/1
  Sum/1 -> Abs/1
  vr/1 -> Sum/1
  Compare To Constant/1 -> Scope1/1, ews_b/1
  v-/1 -> Sum/2

== system Slope_Road_SideSlipAngle_Vx_Estimation/vx estimation/detect overslip // excessive wheel slip(ews)/wheel acceleration deviation criterion ==
  vr : Inport
  ax : Inport  Port=2
  Compare To Constant1 : simulink/Logic and Bit Operations/Compare To Constant  relop=>  const=gao_D_w1  OutDataTypeStr=uint8
  Demux : Demux
  Embedded MATLAB Function : MATLAB Function  TreatAsAtomicUnit=on
  Mux : Mux
  Scope : Scope
  Scope1 : Scope
  Scope2 : Scope
  Scope3 : Scope  NumInputPorts=2
  gao.ay1 : Constant  Value=gao_D_w1
  车轮加速度1 : Subsystem  TreatAsAtomicUnit=on
  车轮加速度2 : Subsystem  TreatAsAtomicUnit=on
  车轮加速度3 : Subsystem  TreatAsAtomicUnit=on
  车轮加速度4 : Subsystem  TreatAsAtomicUnit=on
  ews_c : Outport
  wires:
  车轮加速度2/1(wheel_acc_error) -> Mux/2
  车轮加速度3/1(wheel_acc_error) -> Mux/3
  车轮加速度4/1(wheel_acc_error) -> Mux/4
  Demux/3 -> 车轮加速度3/1(wheel_velo_CoG)
  ax/1 -> 车轮加速度3/2(ax_ms2), 车轮加速度1/2(ax_ms2), 车轮加速度2/2(ax_ms2), 车轮加速度4/2(ax_ms2)
  车轮加速度1/1(wheel_acc_error) -> Mux/1
  Demux/2 -> 车轮加速度2/1(wheel_velo_CoG)
  Demux/4 -> 车轮加速度4/1(wheel_velo_CoG)
  Demux/1 -> 车轮加速度1/1(wheel_velo_CoG)
  vr/1 -> Demux/1
  gao.ay1/1 -> Embedded MATLAB Function/2(gao_D_w1)
  Mux/1 -> Scope/1, Scope3/1, Embedded MATLAB Function/1(u)
  Embedded MATLAB Function/1(y) -> Scope3/2, Compare To Constant1/1
  Compare To Constant1/1 -> Scope1/1, ews_c/1
  Embedded MATLAB Function/2(p) -> Scope2/1

== system Slope_Road_SideSlipAngle_Vx_Estimation/vx estimation/detect overslip // excessive wheel slip(ews)/wheel speed change criterion ==
  vr : Inport
  Abs1 : Abs  SaturateOnIntegerOverflow=off
  Compare To Constant : simulink/Logic and Bit Operations/Compare To Constant  relop=>  const=gao_D_w  OutDataTypeStr=uint8
  Discrete FIR Filter1 : DiscreteFir  Coefficients=delay_constant  AccumDataTypeStr=Inherit: Same as product output
  Embedded MATLAB Function : MATLAB Function  TreatAsAtomicUnit=on
  Scope : Scope
  Scope1 : Scope
  Sum : Sum  Inputs=|+-
  gao.D_w : Constant  Value=gao_D_w
  ews_a : Outport
  wires:
  Embedded MATLAB Function/1(y) -> Compare To Constant/1
  gao.D_w/1 -> Embedded MATLAB Function/2(gao_D_w)
  Sum/1 -> Abs1/1
  Discrete FIR Filter1/1 -> Sum/2
  vr/1 -> Sum/1, Discrete FIR Filter1/1
  Compare To Constant/1 -> Scope1/1, ews_a/1
  Abs1/1 -> Scope/1, Embedded MATLAB Function/1(u)

== system Slope_Road_SideSlipAngle_Vx_Estimation/vx estimation/front_rear_drive process/Atomic Subsystem ==
  vx : Inport
  bestwheel : Inport  Port=2
  ax : Inport  Port=3
  Abs1 : Abs  SaturateOnIntegerOverflow=off
  Add : Sum
  Constant : Constant  Value=Ts
  Constant1 : Constant  Value=-k_vx_vari_thres1
  Constant2 : Constant  Value=-k_vx_vari_thres2
  Constant3 : Constant  Value=-k_vx_vari_thres3
  Constant4 : Constant  Value=ax_vx_thres1
  Constant5 : Constant  Value=ax_vx_thres2
  Constant6 : Constant  Value=0
  Delay : Delay  DelayLength=1  InitialConditionSource=Input port
      settings: InputPortMap=u0,p4
  MATLAB Function : MATLAB Function  TreatAsAtomicUnit=on
  Product : Product
  Product1 : Product
  Subtract : Sum  Inputs=+-
  Switch1 : Switch  Threshold=vx_lowest  SaturateOnIntegerOverflow=off  InputSameDT=off
  vx_esti : Outport
  wires:
  bestwheel/1 -> Delay/2
  vx/1 -> Subtract/2
  Subtract/1 -> Product/1
  Product/1 -> Product1/2
  Constant/1 -> Product1/1
  Product1/1 -> Add/2
  Add/1 -> Delay/1
  ax/1 -> MATLAB Function/1(ax)
  Constant1/1 -> MATLAB Function/4(k_vx_vari_thres1)
  Constant3/1 -> MATLAB Function/6(k_vx_vari_thres3)
  Constant2/1 -> MATLAB Function/5(k_vx_vari_thres2)
  Constant4/1 -> MATLAB Function/2(ax_vx_thres1)
  Constant5/1 -> MATLAB Function/3(ax_vx_thres2)
  MATLAB Function/1(y) -> Product/2
  Switch1/1 -> vx_esti/1
  Delay/1 -> Subtract/1, Add/1, Abs1/1, Switch1/1
  Constant6/1 -> Switch1/3
  Abs1/1 -> Switch1/2

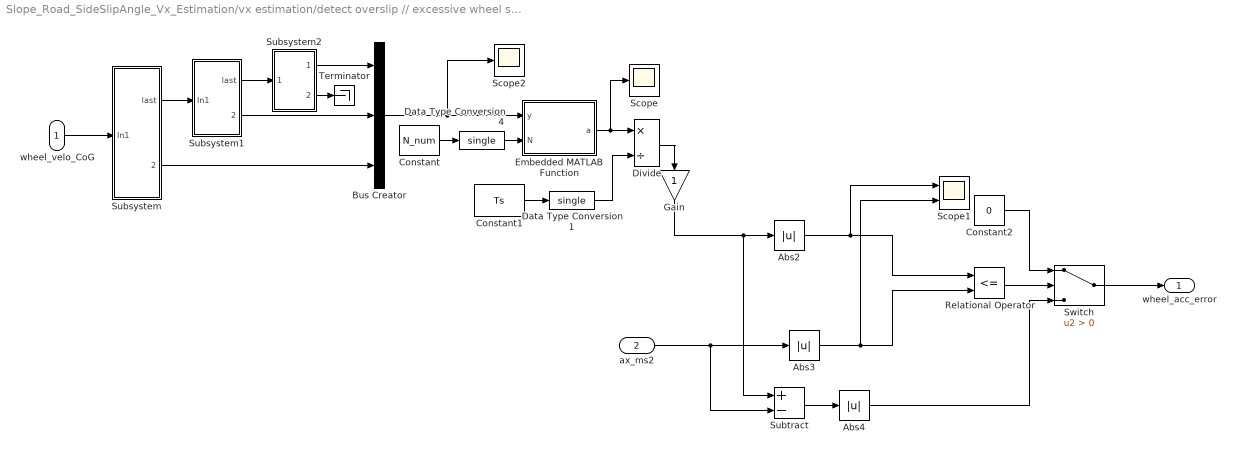
== system Slope_Road_SideSlipAngle_Vx_Estimation/vx estimation/detect overslip // excessive wheel slip(ews)/wheel acceleration deviation criterion/车轮加速度1 ==
  wheel_velo_CoG : Inport
  ax_ms2 : Inport  Port=2
  Abs2 : Abs  SaturateOnIntegerOverflow=off
  Abs3 : Abs  SaturateOnIntegerOverflow=off
  Abs4 : Abs  SaturateOnIntegerOverflow=off
  Bus Creator : BusCreator  Inputs=3
  Constant : Constant  Value=N_num
  Constant1 : Constant  Value=Ts
  Constant2 : Constant  Value=0
  Data Type Conversion1 : DataTypeConversion  OutDataTypeStr=single  SaturateOnIntegerOverflow=off  RndMeth=Floor
  Data Type Conversion4 : DataTypeConversion  OutDataTypeStr=single  SaturateOnIntegerOverflow=off  RndMeth=Floor
  Divide : Product  Inputs=*/
  Embedded MATLAB Function : MATLAB Function  TreatAsAtomicUnit=on
  Gain : Gain
  Relational Operator : RelationalOperator  Operator=<=  OutDataTypeStr=boolean  InputSameDT=off
  Scope : Scope
  Scope1 : Scope  NumInputPorts=2
  Scope2 : Scope
  Subsystem : Subsystem
  Subsystem1 : Subsystem
  Subsystem2 : Subsystem
  Subtract : Sum  Inputs=+-
  Switch : Switch  Criteria=u2 > Threshold  SaturateOnIntegerOverflow=off  InputSameDT=off
  Terminator : Terminator
  wheel_acc_error : Outport
  wires:
  Gain/1 -> Subtract/1, Abs2/1
  Switch/1 -> wheel_acc_error/1
  ax_ms2/1 -> Abs3/1, Subtract/2
  Abs2/1 -> Relational Operator/1, Scope1/1
  Relational Operator/1 -> Switch/2
  Abs3/1 -> Relational Operator/2, Scope1/2
  Subtract/1 -> Abs4/1
  Abs4/1 -> Switch/3
  Constant2/1 -> Switch/1
  Divide/1 -> Gain/1
  wheel_velo_CoG/1 -> Subsystem/1(In1)
  Subsystem1/2(Out1) -> Bus Creator/2
  Subsystem2/1(last) -> Bus Creator/1
  Embedded MATLAB Function/1(a) -> Scope/1, Divide/1
  Subsystem1/1(last) -> Subsystem2/1(In1)
  Bus Creator/1 -> Embedded MATLAB Function/1(y), Scope2/1
  Subsystem/1(last) -> Subsystem1/1(In1)
  Constant/1 -> Data Type Conversion4/1
  Subsystem2/2(Out1) -> Terminator/1
  Subsystem/2(Out1) -> Bus Creator/3
  Constant1/1 -> Data Type Conversion1/1
  Data Type Conversion4/1 -> Embedded MATLAB Function/2(N)
  Data Type Conversion1/1 -> Divide/2

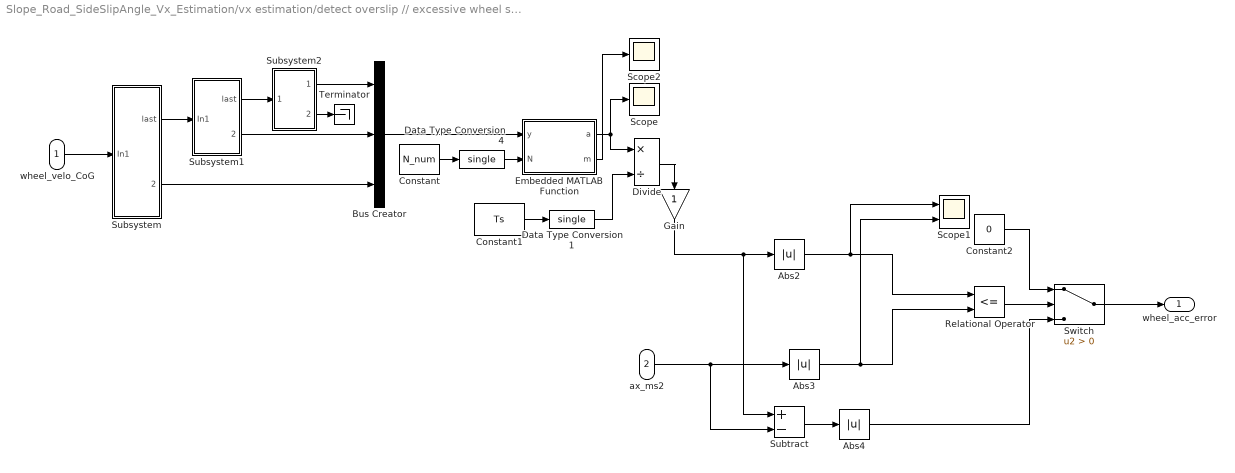
== system Slope_Road_SideSlipAngle_Vx_Estimation/vx estimation/detect overslip // excessive wheel slip(ews)/wheel acceleration deviation criterion/车轮加速度2 ==
  wheel_velo_CoG : Inport
  ax_ms2 : Inport  Port=2
  Abs2 : Abs  SaturateOnIntegerOverflow=off
  Abs3 : Abs  SaturateOnIntegerOverflow=off
  Abs4 : Abs  SaturateOnIntegerOverflow=off
  Bus Creator : BusCreator  Inputs=3
  Constant : Constant  Value=N_num
  Constant1 : Constant  Value=Ts
  Constant2 : Constant  Value=0
  Data Type Conversion1 : DataTypeConversion  OutDataTypeStr=single  SaturateOnIntegerOverflow=off  RndMeth=Floor
  Data Type Conversion4 : DataTypeConversion  OutDataTypeStr=single  SaturateOnIntegerOverflow=off  RndMeth=Floor
  Divide : Product  Inputs=*/
  Embedded MATLAB Function : MATLAB Function  TreatAsAtomicUnit=on
  Gain : Gain
  Relational Operator : RelationalOperator  Operator=<=  OutDataTypeStr=boolean  InputSameDT=off
  Scope : Scope
  Scope1 : Scope  NumInputPorts=2
  Scope2 : Scope
  Subsystem : Subsystem
  Subsystem1 : Subsystem
  Subsystem2 : Subsystem
  Subtract : Sum  Inputs=+-
  Switch : Switch  Criteria=u2 > Threshold  SaturateOnIntegerOverflow=off  InputSameDT=off
  Terminator : Terminator
  wheel_acc_error : Outport
  wires:
  Embedded MATLAB Function/2(m) -> Scope2/1
  Data Type Conversion1/1 -> Divide/2
  Data Type Conversion4/1 -> Embedded MATLAB Function/2(N)
  Constant1/1 -> Data Type Conversion1/1
  Subsystem/2(Out1) -> Bus Creator/3
  Subsystem2/2(Out1) -> Terminator/1
  Constant/1 -> Data Type Conversion4/1
  Subsystem/1(last) -> Subsystem1/1(In1)
  Bus Creator/1 -> Embedded MATLAB Function/1(y)
  Subsystem1/1(last) -> Subsystem2/1(In1)
  Embedded MATLAB Function/1(a) -> Scope/1, Divide/1
  Subsystem2/1(last) -> Bus Creator/1
  Subsystem1/2(Out1) -> Bus Creator/2
  wheel_velo_CoG/1 -> Subsystem/1(In1)
  Divide/1 -> Gain/1
  Constant2/1 -> Switch/1
  Abs4/1 -> Switch/3
  Subtract/1 -> Abs4/1
  Abs3/1 -> Scope1/2, Relational Operator/2
  Relational Operator/1 -> Switch/2
  Abs2/1 -> Scope1/1, Relational Operator/1
  ax_ms2/1 -> Subtract/2, Abs3/1
  Switch/1 -> wheel_acc_error/1
  Gain/1 -> Abs2/1, Subtract/1

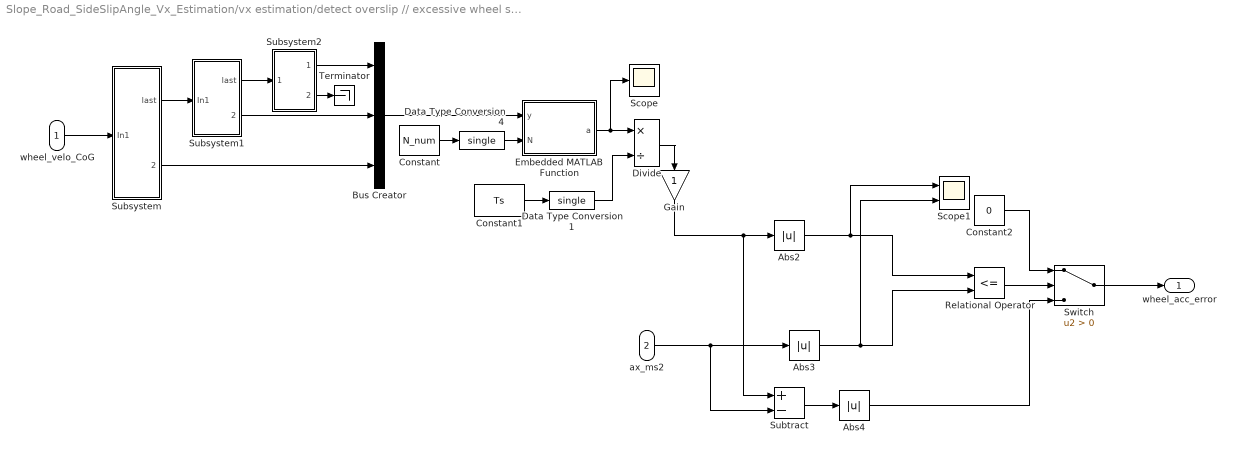
== system Slope_Road_SideSlipAngle_Vx_Estimation/vx estimation/detect overslip // excessive wheel slip(ews)/wheel acceleration deviation criterion/车轮加速度3 ==
  wheel_velo_CoG : Inport
  ax_ms2 : Inport  Port=2
  Abs2 : Abs  SaturateOnIntegerOverflow=off
  Abs3 : Abs  SaturateOnIntegerOverflow=off
  Abs4 : Abs  SaturateOnIntegerOverflow=off
  Bus Creator : BusCreator  Inputs=3
  Constant : Constant  Value=N_num
  Constant1 : Constant  Value=Ts
  Constant2 : Constant  Value=0
  Data Type Conversion1 : DataTypeConversion  OutDataTypeStr=single  SaturateOnIntegerOverflow=off  RndMeth=Floor
  Data Type Conversion4 : DataTypeConversion  OutDataTypeStr=single  SaturateOnIntegerOverflow=off  RndMeth=Floor
  Divide : Product  Inputs=*/
  Embedded MATLAB Function : MATLAB Function  TreatAsAtomicUnit=on
  Gain : Gain
  Relational Operator : RelationalOperator  Operator=<=  OutDataTypeStr=boolean  InputSameDT=off
  Scope : Scope
  Scope1 : Scope  NumInputPorts=2
  Subsystem : Subsystem
  Subsystem1 : Subsystem
  Subsystem2 : Subsystem
  Subtract : Sum  Inputs=+-
  Switch : Switch  Criteria=u2 > Threshold  SaturateOnIntegerOverflow=off  InputSameDT=off
  Terminator : Terminator
  wheel_acc_error : Outport
  wires:
  Gain/1 -> Subtract/1, Abs2/1
  Switch/1 -> wheel_acc_error/1
  ax_ms2/1 -> Abs3/1, Subtract/2
  Abs2/1 -> Relational Operator/1, Scope1/1
  Relational Operator/1 -> Switch/2
  Abs3/1 -> Relational Operator/2, Scope1/2
  Subtract/1 -> Abs4/1
  Abs4/1 -> Switch/3
  Constant2/1 -> Switch/1
  Divide/1 -> Gain/1
  wheel_velo_CoG/1 -> Subsystem/1(In1)
  Subsystem1/2(Out1) -> Bus Creator/2
  Subsystem2/1(last) -> Bus Creator/1
  Embedded MATLAB Function/1(a) -> Scope/1, Divide/1
  Subsystem1/1(last) -> Subsystem2/1(In1)
  Bus Creator/1 -> Embedded MATLAB Function/1(y)
  Subsystem/1(last) -> Subsystem1/1(In1)
  Constant/1 -> Data Type Conversion4/1
  Subsystem2/2(Out1) -> Terminator/1
  Subsystem/2(Out1) -> Bus Creator/3
  Constant1/1 -> Data Type Conversion1/1
  Data Type Conversion4/1 -> Embedded MATLAB Function/2(N)
  Data Type Conversion1/1 -> Divide/2

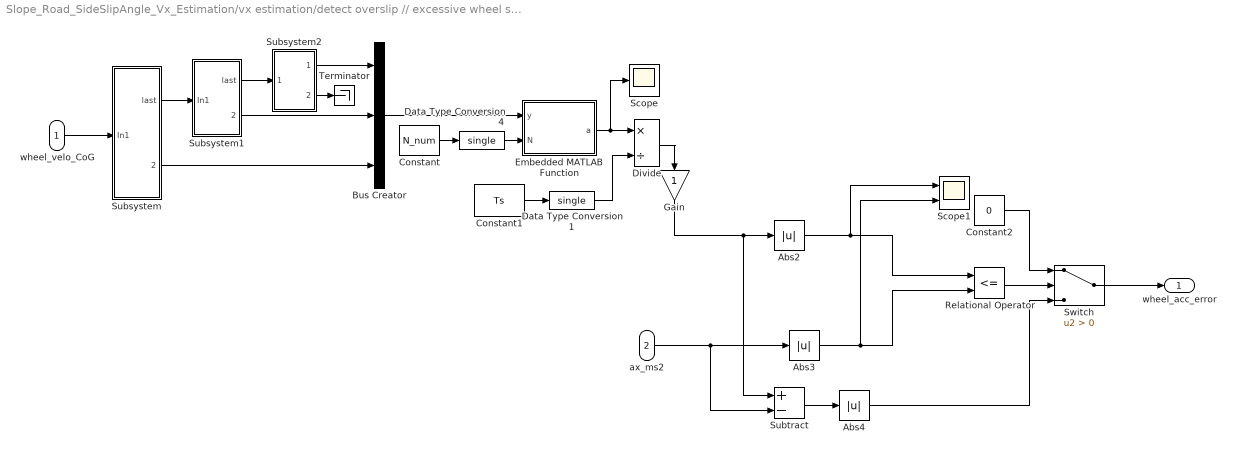
== system Slope_Road_SideSlipAngle_Vx_Estimation/vx estimation/detect overslip // excessive wheel slip(ews)/wheel acceleration deviation criterion/车轮加速度4 ==
  wheel_velo_CoG : Inport
  ax_ms2 : Inport  Port=2
  Abs2 : Abs  SaturateOnIntegerOverflow=off
  Abs3 : Abs  SaturateOnIntegerOverflow=off
  Abs4 : Abs  SaturateOnIntegerOverflow=off
  Bus Creator : BusCreator  Inputs=3
  Constant : Constant  Value=N_num
  Constant1 : Constant  Value=Ts
  Constant2 : Constant  Value=0
  Data Type Conversion1 : DataTypeConversion  OutDataTypeStr=single  SaturateOnIntegerOverflow=off  RndMeth=Floor
  Data Type Conversion4 : DataTypeConversion  OutDataTypeStr=single  SaturateOnIntegerOverflow=off  RndMeth=Floor
  Divide : Product  Inputs=*/
  Embedded MATLAB Function : MATLAB Function  TreatAsAtomicUnit=on
  Gain : Gain
  Relational Operator : RelationalOperator  Operator=<=  OutDataTypeStr=boolean  InputSameDT=off
  Scope : Scope
  Scope1 : Scope  NumInputPorts=2
  Subsystem : Subsystem
  Subsystem1 : Subsystem
  Subsystem2 : Subsystem
  Subtract : Sum  Inputs=+-
  Switch : Switch  Criteria=u2 > Threshold  SaturateOnIntegerOverflow=off  InputSameDT=off
  Terminator : Terminator
  wheel_acc_error : Outport
  wires:
  Data Type Conversion1/1 -> Divide/2
  Data Type Conversion4/1 -> Embedded MATLAB Function/2(N)
  Constant1/1 -> Data Type Conversion1/1
  Subsystem/2(Out1) -> Bus Creator/3
  Subsystem2/2(Out1) -> Terminator/1
  Constant/1 -> Data Type Conversion4/1
  Subsystem/1(last) -> Subsystem1/1(In1)
  Bus Creator/1 -> Embedded MATLAB Function/1(y)
  Subsystem1/1(last) -> Subsystem2/1(In1)
  Embedded MATLAB Function/1(a) -> Divide/1, Scope/1
  Subsystem2/1(last) -> Bus Creator/1
  Subsystem1/2(Out1) -> Bus Creator/2
  wheel_velo_CoG/1 -> Subsystem/1(In1)
  Divide/1 -> Gain/1
  Constant2/1 -> Switch/1
  Abs4/1 -> Switch/3
  Subtract/1 -> Abs4/1
  Abs3/1 -> Scope1/2, Relational Operator/2
  Relational Operator/1 -> Switch/2
  Abs2/1 -> Scope1/1, Relational Operator/1
  ax_ms2/1 -> Subtract/2, Abs3/1
  Switch/1 -> wheel_acc_error/1
  Gain/1 -> Abs2/1, Subtract/1

== system Slope_Road_SideSlipAngle_Vx_Estimation/vx estimation/detect overslip // excessive wheel slip(ews)/wheel acceleration deviation criterion/车轮加速度1/Subsystem ==
  In1 : Inport
  Mux : Mux  Inputs=10
  Unit Delay{,1..8} (9 alike) : UnitDelay  SampleTime=-1  HasFrameUpgradeWarning=on
  last : Outport
  Out1 : Outport  Port=2
  wires:
  Mux/1 -> Out1/1
  In1/1 -> Unit Delay/1, Mux/10
  Unit Delay8/1 -> last/1, Mux/1
  Unit Delay7/1 -> Unit Delay8/1, Mux/2
  Unit Delay6/1 -> Unit Delay7/1, Mux/3
  Unit Delay5/1 -> Unit Delay6/1, Mux/4
  Unit Delay4/1 -> Unit Delay5/1, Mux/5
  Unit Delay3/1 -> Unit Delay4/1, Mux/6
  Unit Delay1/1 -> Unit Delay2/1, Mux/8
  Unit Delay2/1 -> Unit Delay3/1, Mux/7
  Unit Delay/1 -> Unit Delay1/1, Mux/9

== system Slope_Road_SideSlipAngle_Vx_Estimation/vx estimation/detect overslip // excessive wheel slip(ews)/wheel acceleration deviation criterion/车轮加速度1/Subsystem1 ==
  In1 : Inport
  Mux : Mux  Inputs=10
  Unit Delay{1..9} (9 alike) : UnitDelay  SampleTime=-1  HasFrameUpgradeWarning=on
  last : Outport
  Out1 : Outport  Port=2
  wires:
  Unit Delay3/1 -> Unit Delay1/1, Mux/9
  Unit Delay2/1 -> Unit Delay4/1, Mux/7
  Unit Delay1/1 -> Unit Delay2/1, Mux/8
  Unit Delay4/1 -> Unit Delay5/1, Mux/6
  Unit Delay5/1 -> Unit Delay6/1, Mux/5
  Unit Delay6/1 -> Unit Delay7/1, Mux/4
  Unit Delay7/1 -> Unit Delay8/1, Mux/3
  Unit Delay8/1 -> Unit Delay9/1, Mux/2
  Unit Delay9/1 -> Mux/1, last/1
  In1/1 -> Unit Delay3/1, Mux/10
  Mux/1 -> Out1/1

== system Slope_Road_SideSlipAngle_Vx_Estimation/vx estimation/detect overslip // excessive wheel slip(ews)/wheel acceleration deviation criterion/车轮加速度1/Subsystem2 ==
  In1 : Inport
  Mux : Mux  Inputs=10
  Unit Delay{1..9} (9 alike) : UnitDelay  SampleTime=-1  HasFrameUpgradeWarning=on
  last : Outport
  Out1 : Outport  Port=2
  wires:
  Mux/1 -> Out1/1
  In1/1 -> Unit Delay3/1, Mux/10
  Unit Delay9/1 -> last/1, Mux/1
  Unit Delay8/1 -> Unit Delay9/1, Mux/2
  Unit Delay7/1 -> Unit Delay8/1, Mux/3
  Unit Delay6/1 -> Unit Delay7/1, Mux/4
  Unit Delay5/1 -> Unit Delay6/1, Mux/5
  Unit Delay4/1 -> Unit Delay5/1, Mux/6
  Unit Delay1/1 -> Unit Delay2/1, Mux/8
  Unit Delay2/1 -> Unit Delay4/1, Mux/7
  Unit Delay3/1 -> Unit Delay1/1, Mux/9

== system Slope_Road_SideSlipAngle_Vx_Estimation/vx estimation/detect overslip // excessive wheel slip(ews)/wheel acceleration deviation criterion/车轮加速度2/Subsystem ==
  In1 : Inport
  Mux : Mux  Inputs=10
  Unit Delay{,1..8} (9 alike) : UnitDelay  SampleTime=-1  HasFrameUpgradeWarning=on
  last : Outport
  Out1 : Outport  Port=2
  wires:
  Unit Delay/1 -> Mux/9, Unit Delay1/1
  Unit Delay2/1 -> Mux/7, Unit Delay3/1
  Unit Delay1/1 -> Mux/8, Unit Delay2/1
  Unit Delay3/1 -> Mux/6, Unit Delay4/1
  Unit Delay4/1 -> Mux/5, Unit Delay5/1
  Unit Delay5/1 -> Mux/4, Unit Delay6/1
  Unit Delay6/1 -> Mux/3, Unit Delay7/1
  Unit Delay7/1 -> Mux/2, Unit Delay8/1
  Unit Delay8/1 -> Mux/1, last/1
  In1/1 -> Mux/10, Unit Delay/1
  Mux/1 -> Out1/1
